simulink library "casper_library_multipliers"  (Simulink 8.0)
settings: Solver=ode45  SolverMode=SingleTasking  StartTime=0.0  StopTime=10.0  RelTol=1e-3
libraries: xbsIndex_r4 x116
(part 1 of 2)
settings Model: Creator=mdexter  LastModifiedBy=andrew

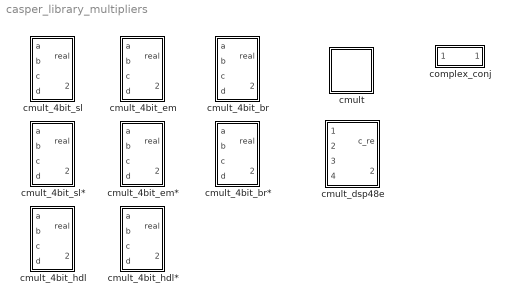
== system casper_library_multipliers ==
  cmult : Subsystem  mask(cmult){n_bits_a=0, bin_pt_a=17, n_bits_b=18, bin_pt_b=17, n_bits_ab=37, bin_pt_ab=14, quantization=Truncate, overflow=Wrap, in_latency=0, mult_latency=3, add_latency=1, conv_latency=1, conjugated=off, async=off, pipelined_enable=on, multiplier_implementation=behavioral HDL}
      mask prompts: n_bits_a "Number of Bits 'a'"; bin_pt_a "Binary Point 'a'"; n_bits_b "Number of Bits 'b'"; bin_pt_b "Binary Point 'b'"; n_bits_ab "Number of Bits 'ab'"; bin_pt_ab "Binary Point 'ab'"; in_latency "Input latency"; mult_latency "Multiplier Latency"; add_latency "Adder Latency"; conv_latency "Convert latency"; conjugated "Conjugate"; async "asynchronous operation"; pipelined_enable "enable pipeline"; multiplier_implementation "Multiplier implementation"
      mask help:
      | Multiplies two complex numbers using 4 multipliers and 2 adders.
      | Conjugation is optional.
      mask init:
      | cmult_init(gcb, ...
      |     'n_bits_a',n_bits_a, ...
      |     'bin_pt_a',bin_pt_a, ...
      |     'n_bits_b',n_bits_b, ...
      |     'bin_pt_b',bin_pt_b, ...
      |     'n_bits_ab',n_bits_ab, ...
      |     'bin_pt_ab',bin_pt_ab, ...
      |     'quantization',quantization, ...
      |     'overflow', overflow, ...
      |     'in_latency', in_latency, ...
      |     'mult_latency', mult_latency, ...
      |     'add_latency', add_latency, ...
      |     'conv_latency', conv_latency, ...
      |     'conjugated', conjugated, ...
      |     'multiplier_implementation', multiplier_implementation, ...
      |     'async', async, ...
      |     'pipelined_enable', pipelined_enable);
      mask TypeOptions quantization: Truncate | Round  (unbiased: +/- Inf) | Round  (unbiased: Even Values)
      mask TypeOptions overflow: Wrap | Saturate | Flag as error
      mask TypeOptions multiplier_implementation: behavioral HDL | standard core | embedded multiplier core
  cmult_4bit_br : Subsystem  mask(cmult_4bit_br){mult_latency=1, add_latency=0}
      mask prompts: mult_latency "Mult Latency"; add_latency "Add Latency"
      mask help: Perform a complex multiplication (a+bi)(c-di)=(ac-bd)+(ad+bc)i. Implements the logic in Block RAM.
      mask Help: eval('xlWeb(''http://casper.berkeley.edu/wiki/Cmult_4bit_br'')')
  cmult_4bit_br* : Subsystem  mask(cmult_4bit_br*){mult_latency=1, add_latency=0}
      mask prompts: mult_latency "Mult Latency"; add_latency "Add Latency"
      mask help: Perform a conjugating complex multiplication (a+bi)(c-di)=(ac+bd)+(bc-ad)i. Implements the logic in Block RAM.
      mask Help: eval('xlWeb(''http://casper.berkeley.edu/wiki/Cmult_4bit_br_'')')
  cmult_4bit_em : Subsystem  mask(cmult_4bit_em){mult_latency=1, add_latency=0}
      mask prompts: mult_latency "Mult Latency"; add_latency "Add Latency"
      mask help: Perform a complex multiplication (a+bi)(c-di)=(ac-bd)+(ad+bc)i. Implements the logic in embedded multipliers.
      mask Help: eval('xlWeb(''http://casper.berkeley.edu/wiki/Cmult_4bit_em'')')
  cmult_4bit_em* : Subsystem  mask(cmult_4bit_em*){mult_latency=1, add_latency=0}
      mask prompts: mult_latency "Mult Latency"; add_latency "Add Latency"
      mask help: Perform a conjugating complex multiplication (a+bi)(c-di)=(ac+bd)+(bc-ad)i. Implements the logic in dedicated multipliers.
      mask Help: eval('xlWeb(''http://casper.berkeley.edu/wiki/Cmult_4bit_em_'')')
  cmult_4bit_hdl : Subsystem  mask(cmult_4bit_sl){mult_latency=1, add_latency=0}
      mask prompts: mult_latency "Mult Latency"; add_latency "Add Latency"
      mask help: Perform a complex multiplication (a+bi)(c-di)=(ac-bd)+(ad+bc)i. Implements the logic in Slices.
      mask Help: eval('xlWeb(''http://casper.berkeley.edu/wiki/Cmult_4bit_sl'')')
  cmult_4bit_hdl* : Subsystem  mask(cmult_4bit_sl*){mult_latency=1, add_latency=0}
      mask prompts: mult_latency "Mult Latency"; add_latency "Add Latency"
      mask help: Perform a conjugating complex multiplication (a+bi)(c-di)=(ac+bd)+(bc-ad)i. Implements the logic in Slices.
      mask Help: eval('xlWeb(''http://casper.berkeley.edu/wiki/Cmult_4bit_sl_'')')
  cmult_4bit_sl : Subsystem  mask(cmult_4bit_sl){mult_latency=1, add_latency=0}
      mask prompts: mult_latency "Mult Latency"; add_latency "Add Latency"
      mask help: Perform a complex multiplication (a+bi)(c-di)=(ac-bd)+(ad+bc)i. Implements the logic in Slices.
      mask Help: eval('xlWeb(''http://casper.berkeley.edu/wiki/Cmult_4bit_sl'')')
  cmult_4bit_sl* : Subsystem  mask(cmult_4bit_sl*){mult_latency=1, add_latency=0}
      mask prompts: mult_latency "Mult Latency"; add_latency "Add Latency"
      mask help: Perform a conjugating complex multiplication (a+bi)(c-di)=(ac+bd)+(bc-ad)i. Implements the logic in Slices.
      mask Help: eval('xlWeb(''http://casper.berkeley.edu/wiki/Cmult_4bit_sl_'')')
  cmult_dsp48e : Subsystem  mask(cmult_dsp48e){n_bits_a=18, bin_pt_a=17, n_bits_b=18, bin_pt_b=17, conjugated=off, full_precision=on, n_bits_c=37, bin_pt_c=34, quantization=Truncate, overflow=Wrap, cast_latency=0}
      mask prompts: n_bits_a "Bit width 'a'"; bin_pt_a "Binary point 'a'"; n_bits_b "Bit width 'b'"; bin_pt_b "Binary point 'b'"; conjugated "Conjugate"; full_precision "Full precision"; n_bits_c "Bit width out"; bin_pt_c "Binary point out"; cast_latency "Cast Latency"
      mask help:
      | Multiplies two complex numbers using 4 DSP48Es.
      | Conjugation is optional.
      |
      | Re{a} and Im{a} can be up to 25 bits.
      | Re{b} and Im{b} can be up to 18 bits.
      mask init:
      | cmult_dsp48e_init(gcb, ...
      |     'n_bits_a', n_bits_a, ...
      |     'bin_pt_a', bin_pt_a, ...
      |     'n_bits_b', n_bits_b, ...
      |     'bin_pt_b', bin_pt_b, ...
      |     'conjugated', conjugated, ...
      |     'full_precision', full_precision, ...
      |     'n_bits_c', n_bits_c, ...
      |     'bin_pt_c', bin_pt_c, ...
      |     'quantization', quantization, ...
      |     'overflow', overflow, ...
      |     'cast_latency', cast_latency);
      settings: AttributesFormatString=|
      | 18_17 * 18_17 ==> 37_34
      | Latency=4
      mask Callback full_precision:
      | full_precision = get_param(gcb, 'full_precision');
      | 
      | if strcmp(full_precision, 'on'),
      |     not_full_precision = 'off';
      | else
      |     not_full_precision = 'on';
      | end
      | 
      | set_param_state(gcb, 'n_bits_c', not_full_precision);
      | set_param_state(gcb, 'bin_pt_c', not_full_precision);
      | set_param_state(gcb, 'quantization', not_full_precision);
      | set_param_state(gcb, 'overflow', not_full_precision);
      | set_param_state(gcb, 'cast_latency', not_full_precision);
      mask TypeOptions quantization: Truncate | Round  (unbiased: +/- Inf) | Round  (unbiased: Even Values)
      mask TypeOptions overflow: Wrap | Saturate | Flag as error
  complex_conj : Subsystem  mask{bitwidth=18, bin_pt=17, latency=3, mode=logic}
      mask prompts: bitwidth "Bit Width"; bin_pt "Binary Point"; mode "Implementation Mode"
      mask init:
      | config.source = str2func('complex_conj_init');
      | config.toplevel = gcb;
      | config.depend = {'complex_conj_init.m'};
      | xBlock( config, {bitwidth, bin_pt, latency, mode});
      mask TypeOptions mode: dsp48e | logic

== system casper_library_multipliers/cmult ==

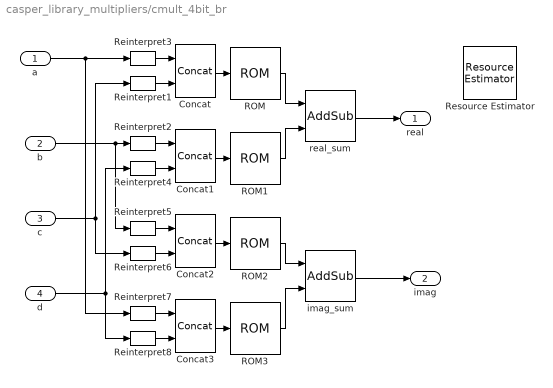
== system casper_library_multipliers/cmult_4bit_br ==
  a : Inport
  b : Inport  Port=2
  c : Inport  Port=3
  d : Inport  Port=4
  Concat{,1..3} (4 alike) : xbsIndex_r4/Concat  num_inputs=2  dbl_ovrd=off  block_type=concat
      settings: block_version=9.1.01
  ROM : xbsIndex_r4/ROM  depth=256  initVector=transpose(transpose([0:7 -8:-1]) * [0:7 -8:-1]) / 64  distributed_mem=Block RAM  rst=off  init_reg=0  en=off  latency=mult_latency  gui_display_data_type=Fixed-point  arith_type="Signed  (2's comp)"  n_bits=8  bin_pt=6  preci_type=Single  exp_width=8  frac_width=24  dbl_ovrd=off  optimize=Area  use_rpm=off  block_type=sprom
      settings: xl_area=[0 0 1 0 0 0 0]
  ROM1 : xbsIndex_r4/ROM  depth=256  initVector=transpose([0:7 -8:-1]) * [0:7 -8:-1] / 64  distributed_mem=Block RAM  rst=off  init_reg=0  en=off  latency=mult_latency  gui_display_data_type=Fixed-point  arith_type="Signed  (2's comp)"  n_bits=8  bin_pt=6  preci_type=Single  exp_width=8  frac_width=24  dbl_ovrd=off  optimize=Area  use_rpm=off  block_type=sprom
      settings: xl_area=[0 0 1 0 0 0 0]
  ROM2 : xbsIndex_r4/ROM  depth=256  initVector=transpose([0:7 -8:-1]) * [0:7 -8:-1] / 64  distributed_mem=Block RAM  rst=off  init_reg=0  en=off  latency=mult_latency  gui_display_data_type=Fixed-point  arith_type="Signed  (2's comp)"  n_bits=8  bin_pt=6  preci_type=Single  exp_width=8  frac_width=24  dbl_ovrd=off  optimize=Area  use_rpm=off  block_type=sprom
      settings: xl_area=[0 0 1 0 0 0 0]
  ROM3 : xbsIndex_r4/ROM  depth=256  initVector=transpose([0:7 -8:-1]) * [0:7 -8:-1] / 64  distributed_mem=Block RAM  rst=off  init_reg=0  en=off  latency=mult_latency  gui_display_data_type=Fixed-point  arith_type="Signed  (2's comp)"  n_bits=8  bin_pt=6  preci_type=Single  exp_width=8  frac_width=24  dbl_ovrd=off  optimize=Area  use_rpm=off  block_type=sprom
      settings: xl_area=[0 0 1 0 0 0 0]
  Reinterpret{1..8} (8 alike) : xbsIndex_r4/Reinterpret  force_arith_type=on  arith_type=Unsigned  force_bin_pt=on  bin_pt=0  block_type=reinterpret
      settings: infoedit="Changes signal type without altering the binary representation.   You can changed the signal between signed and unsigned, and relocate the binary point.<P><P>Hardware notes: In hardware this block costs nothing.<P><P>Example:  Suppose the input is 6 bits wide, signed, with 2 fractional bits, and the output is forced to unsigned with 0 fractional bits.  Then an input of -2.0 (1110.00 in binary 2's complement) becomes an output of 56 (111000 in binary)."  block_version=9.1.01
  Resource Estimator : xbsIndex_r4/Resource Estimator  Tag=resEstTag  Slices=10  FFs=18  BRAMs=4  LUTs=16  IOBs=0  EBMs=0  TBUFs=0  xl_use_estimator_area=off  est_options=Estimate  xl_estimator_area=[10 18 4 16 0 0 0]  mrp_directory=B:\projects\eor_eight_station  simulink_period=1  block_type=resource_estimator
      settings: AttributesFormatString=Resource\nEstimator  block_version=9.1.01
  imag_sum : xbsIndex_r4/AddSub  mode=Addition  use_carryin=off  use_carryout=off  en=off  latency=add_latency  precision=Full  arith_type=Unsigned  n_bits=8  bin_pt=2  quantization=Truncate  overflow=Wrap  dbl_ovrd=off  use_behavioral_HDL=on  hw_selection=Fabric  pipelined=off  use_rpm=on  block_type=addsub
      settings: xl_area=[5 9 0 8 0 0 0]  block_version=9.1.01
  real_sum : xbsIndex_r4/AddSub  mode=Subtraction  use_carryin=off  use_carryout=off  en=off  latency=add_latency  precision=Full  arith_type=Unsigned  n_bits=8  bin_pt=2  quantization=Truncate  overflow=Wrap  dbl_ovrd=off  use_behavioral_HDL=on  hw_selection=Fabric  pipelined=off  use_rpm=on  block_type=addsub
      settings: xl_area=[5 9 0 8 0 0 0]  block_version=9.1.01
  real : Outport
  imag : Outport  Port=2
  wires:
  Reinterpret8/1 -> Concat3/2
  Reinterpret7/1 -> Concat3/1
  Reinterpret6/1 -> Concat2/2
  Reinterpret5/1 -> Concat2/1
  Reinterpret4/1 -> Concat1/2
  Reinterpret2/1 -> Concat1/1
  Reinterpret1/1 -> Concat/2
  Reinterpret3/1 -> Concat/1
  Concat3/1 -> ROM3/1
  Concat2/1 -> ROM2/1
  Concat1/1 -> ROM1/1
  Concat/1 -> ROM/1
  imag_sum/1 -> imag/1
  real_sum/1 -> real/1
  d/1 -> Reinterpret8/1, Reinterpret4/1
  b/1 -> Reinterpret5/1, Reinterpret2/1
  c/1 -> Reinterpret6/1, Reinterpret1/1
  a/1 -> Reinterpret7/1, Reinterpret3/1
  ROM3/1 -> imag_sum/2
  ROM2/1 -> imag_sum/1
  ROM1/1 -> real_sum/2
  ROM/1 -> real_sum/1

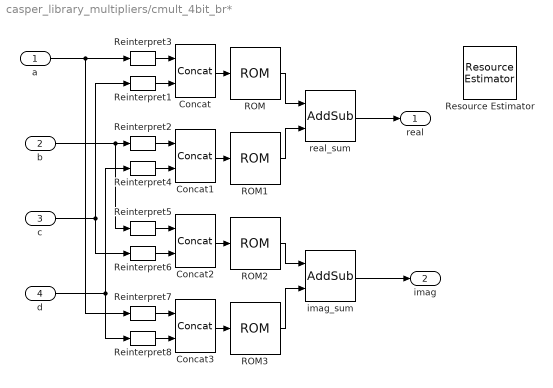
== system casper_library_multipliers/cmult_4bit_br* ==
  a : Inport
  b : Inport  Port=2
  c : Inport  Port=3
  d : Inport  Port=4
  Concat{,1..3} (4 alike) : xbsIndex_r4/Concat  num_inputs=2  dbl_ovrd=off  block_type=concat
      settings: block_version=9.1.01
  ROM : xbsIndex_r4/ROM  depth=256  initVector=transpose(transpose([0:7 -8:-1]) * [0:7 -8:-1]) / 64  distributed_mem=Block RAM  rst=off  init_reg=0  en=off  latency=mult_latency  gui_display_data_type=Fixed-point  arith_type="Signed  (2's comp)"  n_bits=8  bin_pt=6  preci_type=Single  exp_width=8  frac_width=24  dbl_ovrd=off  optimize=Area  use_rpm=off  block_type=sprom
      settings: xl_area=[0 0 1 0 0 0 0]
  ROM1 : xbsIndex_r4/ROM  depth=256  initVector=transpose([0:7 -8:-1]) * [0:7 -8:-1] / 64  distributed_mem=Block RAM  rst=off  init_reg=0  en=off  latency=mult_latency  gui_display_data_type=Fixed-point  arith_type="Signed  (2's comp)"  n_bits=8  bin_pt=6  preci_type=Single  exp_width=8  frac_width=24  dbl_ovrd=off  optimize=Area  use_rpm=off  block_type=sprom
      settings: xl_area=[0 0 1 0 0 0 0]
  ROM2 : xbsIndex_r4/ROM  depth=256  initVector=transpose([0:7 -8:-1]) * [0:7 -8:-1] / 64  distributed_mem=Block RAM  rst=off  init_reg=0  en=off  latency=mult_latency  gui_display_data_type=Fixed-point  arith_type="Signed  (2's comp)"  n_bits=8  bin_pt=6  preci_type=Single  exp_width=8  frac_width=24  dbl_ovrd=off  optimize=Area  use_rpm=off  block_type=sprom
      settings: xl_area=[0 0 1 0 0 0 0]
  ROM3 : xbsIndex_r4/ROM  depth=256  initVector=transpose([0:7 -8:-1]) * [0:7 -8:-1] / 64  distributed_mem=Block RAM  rst=off  init_reg=0  en=off  latency=mult_latency  gui_display_data_type=Fixed-point  arith_type="Signed  (2's comp)"  n_bits=8  bin_pt=6  preci_type=Single  exp_width=8  frac_width=24  dbl_ovrd=off  optimize=Area  use_rpm=off  block_type=sprom
      settings: xl_area=[0 0 1 0 0 0 0]
  Reinterpret{1..8} (8 alike) : xbsIndex_r4/Reinterpret  force_arith_type=on  arith_type=Unsigned  force_bin_pt=on  bin_pt=0  block_type=reinterpret
      settings: infoedit="Changes signal type without altering the binary representation.   You can changed the signal between signed and unsigned, and relocate the binary point.<P><P>Hardware notes: In hardware this block costs nothing.<P><P>Example:  Suppose the input is 6 bits wide, signed, with 2 fractional bits, and the output is forced to unsigned with 0 fractional bits.  Then an input of -2.0 (1110.00 in binary 2's complement) becomes an output of 56 (111000 in binary)."  block_version=9.1.01
  Resource Estimator : xbsIndex_r4/Resource Estimator  Tag=resEstTag  Slices=10  FFs=18  BRAMs=4  LUTs=16  IOBs=0  EBMs=0  TBUFs=0  xl_use_estimator_area=off  est_options=Estimate  xl_estimator_area=[10 18 4 16 0 0 0]  mrp_directory=B:\projects\eor_eight_station  simulink_period=1  block_type=resource_estimator
      settings: AttributesFormatString=Resource\nEstimator  block_version=9.1.01
  imag_sum : xbsIndex_r4/AddSub  mode=Subtraction  use_carryin=off  use_carryout=off  en=off  latency=add_latency  precision=Full  arith_type=Unsigned  n_bits=8  bin_pt=2  quantization=Truncate  overflow=Wrap  dbl_ovrd=off  use_behavioral_HDL=on  hw_selection=Fabric  pipelined=off  use_rpm=on  block_type=addsub
      settings: xl_area=[5 9 0 8 0 0 0]  block_version=9.1.01
  real_sum : xbsIndex_r4/AddSub  mode=Addition  use_carryin=off  use_carryout=off  en=off  latency=add_latency  precision=Full  arith_type=Unsigned  n_bits=8  bin_pt=2  quantization=Truncate  overflow=Wrap  dbl_ovrd=off  use_behavioral_HDL=on  hw_selection=Fabric  pipelined=off  use_rpm=on  block_type=addsub
      settings: xl_area=[5 9 0 8 0 0 0]  block_version=9.1.01
  real : Outport
  imag : Outport  Port=2
  wires:
  ROM/1 -> real_sum/1
  ROM1/1 -> real_sum/2
  ROM2/1 -> imag_sum/1
  ROM3/1 -> imag_sum/2
  a/1 -> Reinterpret3/1, Reinterpret7/1
  c/1 -> Reinterpret1/1, Reinterpret6/1
  b/1 -> Reinterpret2/1, Reinterpret5/1
  d/1 -> Reinterpret4/1, Reinterpret8/1
  real_sum/1 -> real/1
  imag_sum/1 -> imag/1
  Concat/1 -> ROM/1
  Concat1/1 -> ROM1/1
  Concat2/1 -> ROM2/1
  Concat3/1 -> ROM3/1
  Reinterpret3/1 -> Concat/1
  Reinterpret1/1 -> Concat/2
  Reinterpret2/1 -> Concat1/1
  Reinterpret4/1 -> Concat1/2
  Reinterpret5/1 -> Concat2/1
  Reinterpret6/1 -> Concat2/2
  Reinterpret7/1 -> Concat3/1
  Reinterpret8/1 -> Concat3/2

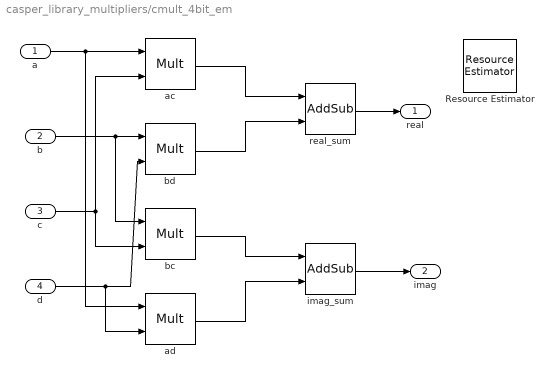
== system casper_library_multipliers/cmult_4bit_em ==
  a : Inport
  b : Inport  Port=2
  c : Inport  Port=3
  d : Inport  Port=4
  Resource Estimator : xbsIndex_r4/Resource Estimator  Tag=resEstTag  Slices=26  FFs=18  BRAMs=0  LUTs=48  IOBs=0  EBMs=4  TBUFs=0  xl_use_estimator_area=off  est_options=Estimate  xl_estimator_area=[26 18 0 48 0 4 0]  mrp_directory=B:\projects\eor_eight_station  simulink_period=1  block_type=resource_estimator
      settings: AttributesFormatString=Resource\nEstimator  block_version=9.1.01
  ac : xbsIndex_r4/Mult  precision=Full  arith_type="Signed  (2's comp)"  n_bits=8  bin_pt=2  quantization=Truncate  overflow=Wrap  en=off  latency=mult_latency  dbl_ovrd=off  use_behavioral_HDL=off  opt=Speed  use_embedded=on  optimum_pipeline=off  pipeline=on  use_rpm=on  placement_style=Rectangular shape  block_type=mult
      settings: infoedit=Hardware notes: To use the internal pipeline stage of the dedicated multiplier you must select 'Pipeline for maximum performance'.  xl_area=[4 0 0 8 0 1 0]  block_version=9.1.01
  ad : xbsIndex_r4/Mult  precision=Full  arith_type="Signed  (2's comp)"  n_bits=8  bin_pt=2  quantization=Truncate  overflow=Wrap  en=off  latency=mult_latency  dbl_ovrd=off  use_behavioral_HDL=off  opt=Speed  use_embedded=on  optimum_pipeline=off  pipeline=on  use_rpm=on  placement_style=Rectangular shape  block_type=mult
      settings: infoedit=Hardware notes: To use the internal pipeline stage of the dedicated multiplier you must select 'Pipeline for maximum performance'.  xl_area=[4 0 0 8 0 1 0]  block_version=9.1.01
  bc : xbsIndex_r4/Mult  precision=Full  arith_type="Signed  (2's comp)"  n_bits=8  bin_pt=2  quantization=Truncate  overflow=Wrap  en=off  latency=mult_latency  dbl_ovrd=off  use_behavioral_HDL=off  opt=Speed  use_embedded=on  optimum_pipeline=off  pipeline=on  use_rpm=on  placement_style=Rectangular shape  block_type=mult
      settings: infoedit=Hardware notes: To use the internal pipeline stage of the dedicated multiplier you must select 'Pipeline for maximum performance'.  xl_area=[4 0 0 8 0 1 0]  block_version=9.1.01
  bd : xbsIndex_r4/Mult  precision=Full  arith_type="Signed  (2's comp)"  n_bits=8  bin_pt=2  quantization=Truncate  overflow=Wrap  en=off  latency=mult_latency  dbl_ovrd=off  use_behavioral_HDL=off  opt=Speed  use_embedded=on  optimum_pipeline=off  pipeline=on  use_rpm=on  placement_style=Rectangular shape  block_type=mult
      settings: infoedit=Hardware notes: To use the internal pipeline stage of the dedicated multiplier you must select 'Pipeline for maximum performance'.  xl_area=[4 0 0 8 0 1 0]  block_version=9.1.01
  imag_sum : xbsIndex_r4/AddSub  mode=Addition  use_carryin=off  use_carryout=off  en=off  latency=add_latency  precision=Full  arith_type=Unsigned  n_bits=8  bin_pt=2  quantization=Truncate  overflow=Wrap  dbl_ovrd=off  use_behavioral_HDL=on  hw_selection=Fabric  pipelined=off  use_rpm=on  block_type=addsub
      settings: xl_area=[5 9 0 8 0 0 0]  block_version=9.1.01
  real_sum : xbsIndex_r4/AddSub  mode=Subtraction  use_carryin=off  use_carryout=off  en=off  latency=add_latency  precision=Full  arith_type=Unsigned  n_bits=8  bin_pt=2  quantization=Truncate  overflow=Wrap  dbl_ovrd=off  use_behavioral_HDL=on  hw_selection=Fabric  pipelined=off  use_rpm=on  block_type=addsub
      settings: xl_area=[5 9 0 8 0 0 0]  block_version=9.1.01
  real : Outport
  imag : Outport  Port=2
  wires:
  imag_sum/1 -> imag/1
  real_sum/1 -> real/1
  d/1 -> bd/2, ad/2
  b/1 -> bd/1, bc/1
  c/1 -> ac/2, bc/2
  a/1 -> ac/1, ad/1
  ad/1 -> imag_sum/2
  bc/1 -> imag_sum/1
  bd/1 -> real_sum/2
  ac/1 -> real_sum/1

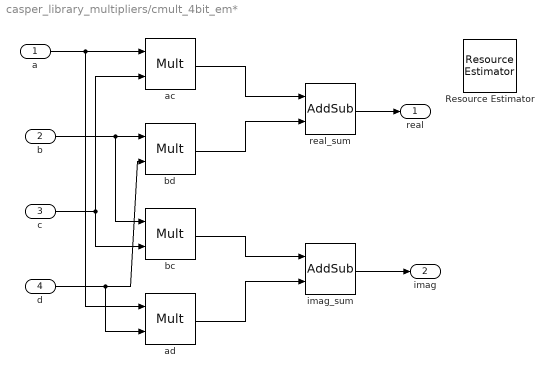
== system casper_library_multipliers/cmult_4bit_em* ==
  a : Inport
  b : Inport  Port=2
  c : Inport  Port=3
  d : Inport  Port=4
  Resource Estimator : xbsIndex_r4/Resource Estimator  Tag=resEstTag  Slices=26  FFs=18  BRAMs=0  LUTs=48  IOBs=0  EBMs=4  TBUFs=0  xl_use_estimator_area=off  est_options=Estimate  xl_estimator_area=[26 18 0 48 0 4 0]  mrp_directory=B:\projects\eor_eight_station  simulink_period=1  block_type=resource_estimator
      settings: AttributesFormatString=Resource\nEstimator  block_version=9.1.01
  ac : xbsIndex_r4/Mult  precision=Full  arith_type="Signed  (2's comp)"  n_bits=8  bin_pt=2  quantization=Truncate  overflow=Wrap  en=off  latency=mult_latency  dbl_ovrd=off  use_behavioral_HDL=off  opt=Speed  use_embedded=on  optimum_pipeline=off  pipeline=on  use_rpm=on  placement_style=Rectangular shape  block_type=mult
      settings: infoedit=Hardware notes: To use the internal pipeline stage of the dedicated multiplier you must select 'Pipeline for maximum performance'.  xl_area=[4 0 0 8 0 1 0]  block_version=9.1.01
  ad : xbsIndex_r4/Mult  precision=Full  arith_type="Signed  (2's comp)"  n_bits=8  bin_pt=2  quantization=Truncate  overflow=Wrap  en=off  latency=mult_latency  dbl_ovrd=off  use_behavioral_HDL=off  opt=Speed  use_embedded=on  optimum_pipeline=off  pipeline=on  use_rpm=on  placement_style=Rectangular shape  block_type=mult
      settings: infoedit=Hardware notes: To use the internal pipeline stage of the dedicated multiplier you must select 'Pipeline for maximum performance'.  xl_area=[4 0 0 8 0 1 0]  block_version=9.1.01
  bc : xbsIndex_r4/Mult  precision=Full  arith_type="Signed  (2's comp)"  n_bits=8  bin_pt=2  quantization=Truncate  overflow=Wrap  en=off  latency=mult_latency  dbl_ovrd=off  use_behavioral_HDL=off  opt=Speed  use_embedded=on  optimum_pipeline=off  pipeline=on  use_rpm=on  placement_style=Rectangular shape  block_type=mult
      settings: infoedit=Hardware notes: To use the internal pipeline stage of the dedicated multiplier you must select 'Pipeline for maximum performance'.  xl_area=[4 0 0 8 0 1 0]  block_version=9.1.01
  bd : xbsIndex_r4/Mult  precision=Full  arith_type="Signed  (2's comp)"  n_bits=8  bin_pt=2  quantization=Truncate  overflow=Wrap  en=off  latency=mult_latency  dbl_ovrd=off  use_behavioral_HDL=off  opt=Speed  use_embedded=on  optimum_pipeline=off  pipeline=on  use_rpm=on  placement_style=Rectangular shape  block_type=mult
      settings: infoedit=Hardware notes: To use the internal pipeline stage of the dedicated multiplier you must select 'Pipeline for maximum performance'.  xl_area=[4 0 0 8 0 1 0]  block_version=9.1.01
  imag_sum : xbsIndex_r4/AddSub  mode=Subtraction  use_carryin=off  use_carryout=off  en=off  latency=add_latency  precision=Full  arith_type=Unsigned  n_bits=8  bin_pt=2  quantization=Truncate  overflow=Wrap  dbl_ovrd=off  use_behavioral_HDL=on  hw_selection=Fabric  pipelined=off  use_rpm=on  block_type=addsub
      settings: xl_area=[5 9 0 8 0 0 0]  block_version=9.1.01
  real_sum : xbsIndex_r4/AddSub  mode=Addition  use_carryin=off  use_carryout=off  en=off  latency=add_latency  precision=Full  arith_type=Unsigned  n_bits=8  bin_pt=2  quantization=Truncate  overflow=Wrap  dbl_ovrd=off  use_behavioral_HDL=on  hw_selection=Fabric  pipelined=off  use_rpm=on  block_type=addsub
      settings: xl_area=[5 9 0 8 0 0 0]  block_version=9.1.01
  real : Outport
  imag : Outport  Port=2
  wires:
  ac/1 -> real_sum/1
  bd/1 -> real_sum/2
  bc/1 -> imag_sum/1
  ad/1 -> imag_sum/2
  a/1 -> ad/1, ac/1
  c/1 -> bc/2, ac/2
  b/1 -> bc/1, bd/1
  d/1 -> ad/2, bd/2
  real_sum/1 -> real/1
  imag_sum/1 -> imag/1

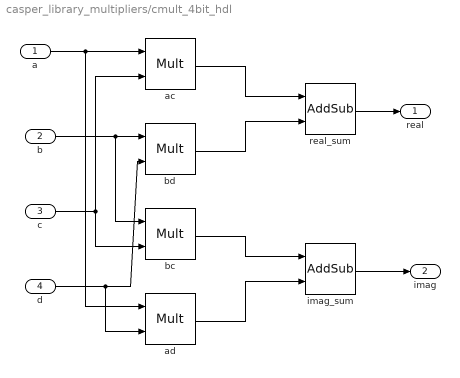
== system casper_library_multipliers/cmult_4bit_hdl ==
  a : Inport
  b : Inport  Port=2
  c : Inport  Port=3
  d : Inport  Port=4
  ac : xbsIndex_r4/Mult  precision=Full  arith_type="Signed  (2's comp)"  n_bits=7  bin_pt=6  quantization=Truncate  overflow=Wrap  en=off  latency=mult_latency  dbl_ovrd=off  use_behavioral_HDL=on  opt=Speed  use_embedded=off  optimum_pipeline=off  pipeline=off  use_rpm=on  placement_style=Rectangular shape  block_type=mult
      settings: infoedit=Hardware notes: To use the internal pipeline stage of the dedicated multiplier you must select 'Pipeline for maximum performance'.  xl_area=[10 7 0 17 0 0 0]  block_version=9.1.01
  ad : xbsIndex_r4/Mult  precision=Full  arith_type="Signed  (2's comp)"  n_bits=7  bin_pt=6  quantization=Truncate  overflow=Wrap  en=off  latency=mult_latency  dbl_ovrd=off  use_behavioral_HDL=on  opt=Speed  use_embedded=off  optimum_pipeline=off  pipeline=off  use_rpm=on  placement_style=Rectangular shape  block_type=mult
      settings: infoedit=Hardware notes: To use the internal pipeline stage of the dedicated multiplier you must select 'Pipeline for maximum performance'.  xl_area=[10 7 0 17 0 0 0]  block_version=9.1.01
  bc : xbsIndex_r4/Mult  precision=Full  arith_type="Signed  (2's comp)"  n_bits=7  bin_pt=6  quantization=Truncate  overflow=Wrap  en=off  latency=mult_latency  dbl_ovrd=off  use_behavioral_HDL=on  opt=Speed  use_embedded=off  optimum_pipeline=off  pipeline=off  use_rpm=on  placement_style=Rectangular shape  block_type=mult
      settings: infoedit=Hardware notes: To use the internal pipeline stage of the dedicated multiplier you must select 'Pipeline for maximum performance'.  xl_area=[10 7 0 17 0 0 0]  block_version=9.1.01
  bd : xbsIndex_r4/Mult  precision=Full  arith_type="Signed  (2's comp)"  n_bits=7  bin_pt=6  quantization=Truncate  overflow=Wrap  en=off  latency=mult_latency  dbl_ovrd=off  use_behavioral_HDL=on  opt=Speed  use_embedded=off  optimum_pipeline=off  pipeline=off  use_rpm=on  placement_style=Rectangular shape  block_type=mult
      settings: infoedit=Hardware notes: To use the internal pipeline stage of the dedicated multiplier you must select 'Pipeline for maximum performance'.  xl_area=[10 7 0 17 0 0 0]  block_version=9.1.01
  imag_sum : xbsIndex_r4/AddSub  mode=Addition  use_carryin=off  use_carryout=off  en=off  latency=add_latency  precision=Full  arith_type=Unsigned  n_bits=8  bin_pt=2  quantization=Truncate  overflow=Wrap  dbl_ovrd=off  use_behavioral_HDL=on  hw_selection=Fabric  pipelined=off  use_rpm=on  block_type=addsub
      settings: xl_area=[4 8 0 7 0 0 0]  block_version=9.1.01
  real_sum : xbsIndex_r4/AddSub  mode=Subtraction  use_carryin=off  use_carryout=off  en=off  latency=add_latency  precision=Full  arith_type=Unsigned  n_bits=8  bin_pt=2  quantization=Truncate  overflow=Wrap  dbl_ovrd=off  use_behavioral_HDL=on  hw_selection=Fabric  pipelined=off  use_rpm=on  block_type=addsub
      settings: xl_area=[4 8 0 7 0 0 0]  block_version=9.1.01
  real : Outport
  imag : Outport  Port=2
  wires:
  imag_sum/1 -> imag/1
  real_sum/1 -> real/1
  d/1 -> bd/2, ad/2
  b/1 -> bd/1, bc/1
  c/1 -> ac/2, bc/2
  a/1 -> ac/1, ad/1
  ad/1 -> imag_sum/2
  bc/1 -> imag_sum/1
  bd/1 -> real_sum/2
  ac/1 -> real_sum/1

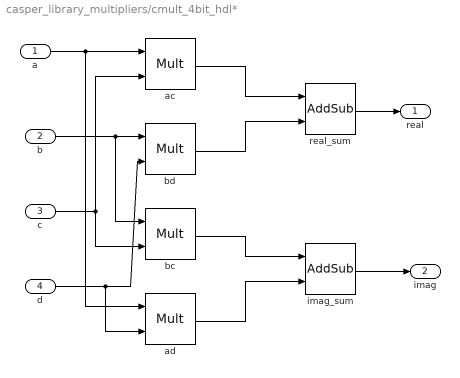
== system casper_library_multipliers/cmult_4bit_hdl* ==
  a : Inport
  b : Inport  Port=2
  c : Inport  Port=3
  d : Inport  Port=4
  ac : xbsIndex_r4/Mult  precision=Full  arith_type="Signed  (2's comp)"  n_bits=7  bin_pt=6  quantization=Truncate  overflow=Wrap  en=off  latency=mult_latency  dbl_ovrd=off  use_behavioral_HDL=on  opt=Speed  use_embedded=off  optimum_pipeline=off  pipeline=off  use_rpm=on  placement_style=Rectangular shape  block_type=mult
      settings: infoedit=Hardware notes: To use the internal pipeline stage of the dedicated multiplier you must select 'Pipeline for maximum performance'.  xl_area=[10 7 0 17 0 0 0]  block_version=9.1.01
  ad : xbsIndex_r4/Mult  precision=Full  arith_type="Signed  (2's comp)"  n_bits=7  bin_pt=6  quantization=Truncate  overflow=Wrap  en=off  latency=mult_latency  dbl_ovrd=off  use_behavioral_HDL=on  opt=Speed  use_embedded=off  optimum_pipeline=off  pipeline=off  use_rpm=on  placement_style=Rectangular shape  block_type=mult
      settings: infoedit=Hardware notes: To use the internal pipeline stage of the dedicated multiplier you must select 'Pipeline for maximum performance'.  xl_area=[10 7 0 17 0 0 0]  block_version=9.1.01
  bc : xbsIndex_r4/Mult  precision=Full  arith_type="Signed  (2's comp)"  n_bits=7  bin_pt=6  quantization=Truncate  overflow=Wrap  en=off  latency=mult_latency  dbl_ovrd=off  use_behavioral_HDL=on  opt=Speed  use_embedded=off  optimum_pipeline=off  pipeline=off  use_rpm=on  placement_style=Rectangular shape  block_type=mult
      settings: infoedit=Hardware notes: To use the internal pipeline stage of the dedicated multiplier you must select 'Pipeline for maximum performance'.  xl_area=[10 7 0 17 0 0 0]  block_version=9.1.01
  bd : xbsIndex_r4/Mult  precision=Full  arith_type="Signed  (2's comp)"  n_bits=7  bin_pt=6  quantization=Truncate  overflow=Wrap  en=off  latency=mult_latency  dbl_ovrd=off  use_behavioral_HDL=on  opt=Speed  use_embedded=off  optimum_pipeline=off  pipeline=off  use_rpm=on  placement_style=Rectangular shape  block_type=mult
      settings: infoedit=Hardware notes: To use the internal pipeline stage of the dedicated multiplier you must select 'Pipeline for maximum performance'.  xl_area=[10 7 0 17 0 0 0]  block_version=9.1.01
  imag_sum : xbsIndex_r4/AddSub  mode=Subtraction  use_carryin=off  use_carryout=off  en=off  latency=add_latency  precision=Full  arith_type=Unsigned  n_bits=8  bin_pt=2  quantization=Truncate  overflow=Wrap  dbl_ovrd=off  use_behavioral_HDL=on  hw_selection=Fabric  pipelined=off  use_rpm=on  block_type=addsub
      settings: xl_area=[4 8 0 7 0 0 0]  block_version=9.1.01
  real_sum : xbsIndex_r4/AddSub  mode=Addition  use_carryin=off  use_carryout=off  en=off  latency=add_latency  precision=Full  arith_type=Unsigned  n_bits=8  bin_pt=2  quantization=Truncate  overflow=Wrap  dbl_ovrd=off  use_behavioral_HDL=on  hw_selection=Fabric  pipelined=off  use_rpm=on  block_type=addsub
      settings: xl_area=[4 8 0 7 0 0 0]  block_version=9.1.01
  real : Outport
  imag : Outport  Port=2
  wires:
  ac/1 -> real_sum/1
  bd/1 -> real_sum/2
  bc/1 -> imag_sum/1
  ad/1 -> imag_sum/2
  a/1 -> ad/1, ac/1
  c/1 -> bc/2, ac/2
  b/1 -> bc/1, bd/1
  d/1 -> ad/2, bd/2
  real_sum/1 -> real/1
  imag_sum/1 -> imag/1

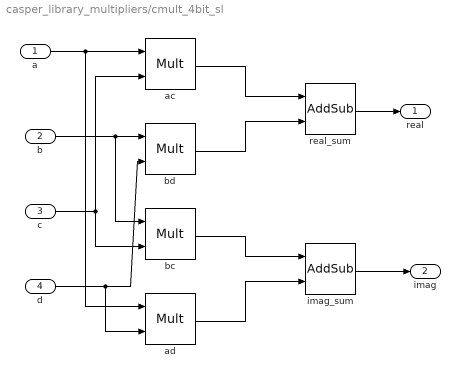
== system casper_library_multipliers/cmult_4bit_sl ==
  a : Inport
  b : Inport  Port=2
  c : Inport  Port=3
  d : Inport  Port=4
  ac : xbsIndex_r4/Mult  precision=Full  arith_type="Signed  (2's comp)"  n_bits=7  bin_pt=6  quantization=Truncate  overflow=Wrap  en=off  latency=mult_latency  dbl_ovrd=off  use_behavioral_HDL=off  opt=Speed  use_embedded=off  optimum_pipeline=off  pipeline=off  use_rpm=on  placement_style=Rectangular shape  block_type=mult
      settings: infoedit=Hardware notes: To use the internal pipeline stage of the dedicated multiplier you must select 'Pipeline for maximum performance'.  xl_area=[10 7 0 17 0 0 0]  block_version=9.1.01
  ad : xbsIndex_r4/Mult  precision=Full  arith_type="Signed  (2's comp)"  n_bits=7  bin_pt=6  quantization=Truncate  overflow=Wrap  en=off  latency=mult_latency  dbl_ovrd=off  use_behavioral_HDL=off  opt=Speed  use_embedded=off  optimum_pipeline=off  pipeline=off  use_rpm=on  placement_style=Rectangular shape  block_type=mult
      settings: infoedit=Hardware notes: To use the internal pipeline stage of the dedicated multiplier you must select 'Pipeline for maximum performance'.  xl_area=[10 7 0 17 0 0 0]  block_version=9.1.01
  bc : xbsIndex_r4/Mult  precision=Full  arith_type="Signed  (2's comp)"  n_bits=7  bin_pt=6  quantization=Truncate  overflow=Wrap  en=off  latency=mult_latency  dbl_ovrd=off  use_behavioral_HDL=off  opt=Speed  use_embedded=off  optimum_pipeline=off  pipeline=off  use_rpm=on  placement_style=Rectangular shape  block_type=mult
      settings: infoedit=Hardware notes: To use the internal pipeline stage of the dedicated multiplier you must select 'Pipeline for maximum performance'.  xl_area=[10 7 0 17 0 0 0]  block_version=9.1.01
  bd : xbsIndex_r4/Mult  precision=Full  arith_type="Signed  (2's comp)"  n_bits=7  bin_pt=6  quantization=Truncate  overflow=Wrap  en=off  latency=mult_latency  dbl_ovrd=off  use_behavioral_HDL=off  opt=Speed  use_embedded=off  optimum_pipeline=off  pipeline=off  use_rpm=on  placement_style=Rectangular shape  block_type=mult
      settings: infoedit=Hardware notes: To use the internal pipeline stage of the dedicated multiplier you must select 'Pipeline for maximum performance'.  xl_area=[10 7 0 17 0 0 0]  block_version=9.1.01
  imag_sum : xbsIndex_r4/AddSub  mode=Addition  use_carryin=off  use_carryout=off  en=off  latency=add_latency  precision=Full  arith_type=Unsigned  n_bits=8  bin_pt=2  quantization=Truncate  overflow=Wrap  dbl_ovrd=off  use_behavioral_HDL=on  hw_selection=Fabric  pipelined=off  use_rpm=on  block_type=addsub
      settings: xl_area=[4 8 0 7 0 0 0]  block_version=9.1.01
  real_sum : xbsIndex_r4/AddSub  mode=Subtraction  use_carryin=off  use_carryout=off  en=off  latency=add_latency  precision=Full  arith_type=Unsigned  n_bits=8  bin_pt=2  quantization=Truncate  overflow=Wrap  dbl_ovrd=off  use_behavioral_HDL=on  hw_selection=Fabric  pipelined=off  use_rpm=on  block_type=addsub
      settings: xl_area=[4 8 0 7 0 0 0]  block_version=9.1.01
  real : Outport
  imag : Outport  Port=2
  wires:
  ac/1 -> real_sum/1
  bd/1 -> real_sum/2
  bc/1 -> imag_sum/1
  ad/1 -> imag_sum/2
  a/1 -> ad/1, ac/1
  c/1 -> bc/2, ac/2
  b/1 -> bc/1, bd/1
  d/1 -> ad/2, bd/2
  real_sum/1 -> real/1
  imag_sum/1 -> imag/1

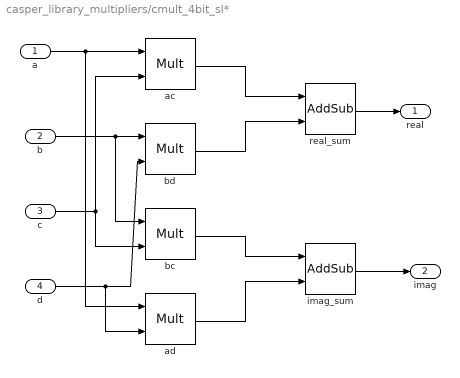
== system casper_library_multipliers/cmult_4bit_sl* ==
  a : Inport
  b : Inport  Port=2
  c : Inport  Port=3
  d : Inport  Port=4
  ac : xbsIndex_r4/Mult  precision=Full  arith_type="Signed  (2's comp)"  n_bits=7  bin_pt=6  quantization=Truncate  overflow=Wrap  en=off  latency=mult_latency  dbl_ovrd=off  use_behavioral_HDL=off  opt=Speed  use_embedded=off  optimum_pipeline=off  pipeline=off  use_rpm=on  placement_style=Rectangular shape  block_type=mult
      settings: infoedit=Hardware notes: To use the internal pipeline stage of the dedicated multiplier you must select 'Pipeline for maximum performance'.  xl_area=[10 7 0 17 0 0 0]  block_version=9.1.01
  ad : xbsIndex_r4/Mult  precision=Full  arith_type="Signed  (2's comp)"  n_bits=7  bin_pt=6  quantization=Truncate  overflow=Wrap  en=off  latency=mult_latency  dbl_ovrd=off  use_behavioral_HDL=off  opt=Speed  use_embedded=off  optimum_pipeline=off  pipeline=off  use_rpm=on  placement_style=Rectangular shape  block_type=mult
      settings: infoedit=Hardware notes: To use the internal pipeline stage of the dedicated multiplier you must select 'Pipeline for maximum performance'.  xl_area=[10 7 0 17 0 0 0]  block_version=9.1.01
  bc : xbsIndex_r4/Mult  precision=Full  arith_type="Signed  (2's comp)"  n_bits=7  bin_pt=6  quantization=Truncate  overflow=Wrap  en=off  latency=mult_latency  dbl_ovrd=off  use_behavioral_HDL=off  opt=Speed  use_embedded=off  optimum_pipeline=off  pipeline=off  use_rpm=on  placement_style=Rectangular shape  block_type=mult
      settings: infoedit=Hardware notes: To use the internal pipeline stage of the dedicated multiplier you must select 'Pipeline for maximum performance'.  xl_area=[10 7 0 17 0 0 0]  block_version=9.1.01
  bd : xbsIndex_r4/Mult  precision=Full  arith_type="Signed  (2's comp)"  n_bits=7  bin_pt=6  quantization=Truncate  overflow=Wrap  en=off  latency=mult_latency  dbl_ovrd=off  use_behavioral_HDL=off  opt=Speed  use_embedded=off  optimum_pipeline=off  pipeline=off  use_rpm=on  placement_style=Rectangular shape  block_type=mult
      settings: infoedit=Hardware notes: To use the internal pipeline stage of the dedicated multiplier you must select 'Pipeline for maximum performance'.  xl_area=[10 7 0 17 0 0 0]  block_version=9.1.01
  imag_sum : xbsIndex_r4/AddSub  mode=Subtraction  use_carryin=off  use_carryout=off  en=off  latency=add_latency  precision=Full  arith_type=Unsigned  n_bits=8  bin_pt=2  quantization=Truncate  overflow=Wrap  dbl_ovrd=off  use_behavioral_HDL=on  hw_selection=Fabric  pipelined=off  use_rpm=on  block_type=addsub
      settings: xl_area=[4 8 0 7 0 0 0]  block_version=9.1.01
  real_sum : xbsIndex_r4/AddSub  mode=Addition  use_carryin=off  use_carryout=off  en=off  latency=add_latency  precision=Full  arith_type=Unsigned  n_bits=8  bin_pt=2  quantization=Truncate  overflow=Wrap  dbl_ovrd=off  use_behavioral_HDL=on  hw_selection=Fabric  pipelined=off  use_rpm=on  block_type=addsub
      settings: xl_area=[4 8 0 7 0 0 0]  block_version=9.1.01
  real : Outport
  imag : Outport  Port=2
  wires:
  imag_sum/1 -> imag/1
  real_sum/1 -> real/1
  d/1 -> bd/2, ad/2
  b/1 -> bd/1, bc/1
  c/1 -> ac/2, bc/2
  a/1 -> ac/1, ad/1
  ad/1 -> imag_sum/2
  bc/1 -> imag_sum/1
  bd/1 -> real_sum/2
  ac/1 -> real_sum/1
